simulink model "LKA_Replay_Harness"  (R2026a)
settings: Solver=FixedStepDiscrete  FixedStep=LKA.Ts
undefined symbols (not defined in the file): LKA
Description:
  | Open-loop replay of LKA_Controller on recorded lane measurements (lka_replay_controller.m): REPLAY.Sensor (LaneSensorBus timeseries), REPLAY.Speed, REPLAY.YawRate.
settings Model: Creator=rithv  LastModifiedBy=rithv

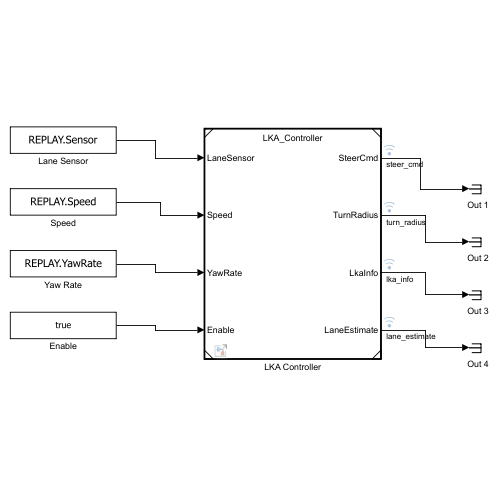
[thumbnail: Simulink's stored preview of the top-level diagram]
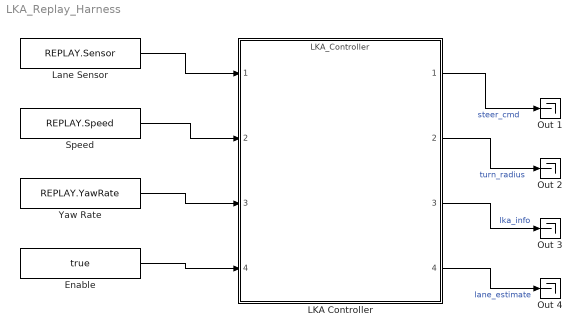
== system LKA_Replay_Harness ==
  Enable : Constant  Value=true  OutDataTypeStr=boolean  SampleTime=LKA.Ts
  LKA Controller : ModelReference  ModelNameDialog=LKA_Controller  SimulationMode=Normal  ModelReferenceVersion=1.1
  Lane Sensor : FromWorkspace  VariableName=REPLAY.Sensor  OutDataTypeStr=Bus: LaneSensorBus  SampleTime=LKA.Ts  Interpolate=off  OutputAfterFinalValue=Holding final value
  Out {1..4} (4 alike) : Terminator
  Speed : FromWorkspace  VariableName=REPLAY.Speed  SampleTime=LKA.Ts  Interpolate=off  OutputAfterFinalValue=Holding final value
  Yaw Rate : FromWorkspace  VariableName=REPLAY.YawRate  SampleTime=LKA.Ts  Interpolate=off  OutputAfterFinalValue=Holding final value
  wires:
  Lane Sensor/1 -> LKA Controller/1
  Speed/1 -> LKA Controller/2
  Yaw Rate/1 -> LKA Controller/3
  Enable/1 -> LKA Controller/4
  LKA Controller/1 -> Out 1/1  "steer_cmd"
  LKA Controller/2 -> Out 2/1  "turn_radius"
  LKA Controller/3 -> Out 3/1  "lka_info"
  LKA Controller/4 -> Out 4/1  "lane_estimate"
